simulink model "ConfiguredHevMmVirtualVehicle"  (R2025b)
settings: configuration reference "VehicleVariable" (kept outside this file)
StartFcn:
  | %tic
StopFcn:
  | %toc
model workspace (MAT data in the model file):
  ExtDrvCmdsSwitch : Simulink.Parameter (value not decoded)
  ExtDrvRefSwitch : Simulink.Parameter (value not decoded)
  ExtEnvSwitch : Simulink.Parameter (value not decoded)
  ExtGndSwitch : Simulink.Parameter (value not decoded)
symbols that are objects in the model workspace (value not decoded): ExtDrvCmdsSwitch, ExtDrvRefSwitch, ExtEnvSwitch, ExtGndSwitch
undefined symbols (not defined in the file or in its folder): AmbTemp, BaroPress, CurvGradRef, CurvRef, DCM, DriverAeroRes, DriverDrivelineRes, DriverInitialGear, DriverPreviewDist, DriverRollRes, DriverShiftTime, DriverTimeConst, DriverTractiveForce, EnvAbsPrs, EnvAirTemp, EnvGrvty, EnvNomFrictionScaling, EnvNominalGrade, EnvScnFrictionMap, EnvScnFrictionMapXBpts, EnvScnFrictionMapYBpts, EnvScnHeightMap, EnvScnHeightMapXBpts, EnvScnHeightMapYBpts, EnvWindVelX, EnvWindVelY, EnvWindVelZ, Gnd, Grade, HazzardCmd, HighBeamCmd, lambda_mux, LeftSignalCmd, LngRef, LowBeamCmd, LtrRef, PhiRef, PlntVehDstCGFrntAxl, PlntVehDstCGRearAxl, PlntVehInitLatPos, PlntVehInitLongPos, PlntVehInitPitchAng, PlntVehInitRollAng, PlntVehInitVertPos, PlntVehInitYawAng, PlntVehMass, PlntVehTrckWdth, PlntVehYawMomentInertia, PlntWhlLdRadiusFrnt, PlntWhlLdRadiusRear, RightSignalCmd, ScnCRRadius, Sim3dSensor, Wind, XRef, YRef, Z
libraries: simulink x28, autolibutils x8, autolibsharedcommon x7, vehdynlibscenariocommon x7, vehdynlibviscommon x4, vehdynlibdriver x2, sim3dgroundtruthsensorlib x2, sim3dlib x2, autolibshared x2, sim3dautolib x2, sl3dlib x1, sharedtransform x1
(part 4 of 6)

== system ConfiguredHevMmVirtualVehicle/Scenarios/Reference Generator/Constant Radius ==
  VehFdbk : Inport
  Bus Creator : BusCreator  Inputs=3
  Bus Selector : BusSelector  OutputSignals=Body.InertFrm.Geom.Disp.Z,Body.InertFrm.Geom.Disp.X,Body.InertFrm.Geom.Disp.Y,Body.InertFrm.Cg.Ang.psi
  Bus Selector1 : BusSelector  OutputSignals=XRef,YRef
  Constant Radius : vehdynlibscenariocommon/Constant Radius Signal Input  VariantControl=4  tStart=ScnStartTime  velRef=ScnLongVelRef  velRefUnit=mph  R=ScnCRRadius  X_o=PlntVehInitLongPos  Y_o=PlntVehInitLatPos  psi_o=PlntVehInitYawAng  radialConeDist=6  ayMax=ScnCRMaxLatAccel  steerDir=Right  ayStop=off  use3DCones=off  aMode=2
      settings: LibrarySourceBlock=vehdynlibscenario/Constant Radius
  Signal Copy : SignalConversion  OverrideOpt=off
  Signal Copy1 : SignalConversion  OverrideOpt=off
  Signal Copy2 : SignalConversion  OverrideOpt=off
  " Vis" : Outport
  DrvRef : Outport  Port=2  VectorParamsAs1DForOutWhenUnconnected=off
  DrvCmd : Outport  Port=3  VectorParamsAs1DForOutWhenUnconnected=off
  " Fdbk" : Outport  Port=4  VectorParamsAs1DForOutWhenUnconnected=off
  wires:
  VehFdbk/1 -> " Fdbk"/1, Bus Selector/1
  Bus Creator/1 -> " Vis"/1
  Constant Radius/2 -> DrvCmd/1
  Bus Selector/2 -> Constant Radius/1  "<X>"
  Bus Selector/3 -> Constant Radius/2  "<Y>"
  Bus Selector/4 -> Constant Radius/3  "<psi>"
  Constant Radius/1 -> Bus Selector1/1, DrvRef/1
  Bus Selector/1 -> Signal Copy/1  "<Z>"
  Signal Copy/1 -> Bus Creator/3  "ZRef"
  Signal Copy1/1 -> Bus Creator/2  "YRef"
  Signal Copy2/1 -> Bus Creator/1  "XRef"
  Bus Selector1/2 -> Signal Copy1/1  "<YRef>"
  Bus Selector1/1 -> Signal Copy2/1  "<XRef>"

== system ConfiguredHevMmVirtualVehicle/Scenarios/Reference Generator/Double Lane Change ==
  "VehFdbk " : Inport
  Bus Selector : BusSelector  OutputSignals=Body.BdyFrm.Cg.Vel.xdot,Body.InertFrm.Geom.Disp.X,Body.InertFrm.Geom.Disp.Y,Body.InertFrm.Cg.Ang.psi
  Double Lane Change : vehdynlibscenariocommon/Lane Change Signal Input  ssMode=Initialize from model  ssVar=dlcSS35mph  changeType=Obstacle avoidance (ISO 3888-2)  tStart=ScnStartTime  XGate=ScnDLCGateLongPos  velRef=ScnLongVelRef  velRefUnit=mph  xStart=ScnDLCLongRefStartPos  vehWidth=ScnDLCVehicleWidth  nomLatOffset=ScnDLCLatRefOffset  latRefbp=ScnDLCLongRefBpt  latRef=ScnDLCLatRef  centerSwitch=on  xSimStop=off  extInfo=on  use3DCones=off  ssDefault=on  X_o=0  Y_o=3.125  psi_o=0  ssTol=.1  ssMaxTime=30  ssWSName=dlcSS35mph  aMode=2
      settings: LibrarySourceBlock=vehdynlibscenario/Lane Change
  " Vis" : Outport  VectorParamsAs1DForOutWhenUnconnected=off
  DrvRef : Outport  Port=2  VectorParamsAs1DForOutWhenUnconnected=off
  DrvCmd : Outport  Port=3  VectorParamsAs1DForOutWhenUnconnected=off
  " Fdbk" : Outport  Port=4  VectorParamsAs1DForOutWhenUnconnected=off
  wires:
  "VehFdbk "/1 -> " Fdbk"/1, Bus Selector/1
  Double Lane Change/1 -> " Vis"/1
  Double Lane Change/2 -> DrvRef/1
  Bus Selector/1 -> Double Lane Change/1  "<xdot>"
  Double Lane Change/3 -> DrvCmd/1
  Bus Selector/2 -> Double Lane Change/2  "<X>"
  Bus Selector/3 -> Double Lane Change/3  "<Y>"
  Bus Selector/4 -> Double Lane Change/4  "<psi>"

== system ConfiguredHevMmVirtualVehicle/Scenarios/Reference Generator/Drive Cycle ==
  "VehFdbk " : Inport
  Bus Assignment : BusAssignment  AssignedSignals=LngRef,XRef
  Bus Creator : BusCreator  Inputs=3
  Bus Selector : BusSelector  OutputSignals=Body.InertFrm.Cg.Disp.X
  Constant13 : Constant  Value=0
  Constant14 : Constant  Value=0
  Constant15 : Constant  Value=0
  Drive Cycle Source : autolibshared/Drive Cycle Source  cycleVar=FTP75  fileVar=L:\Bauto\matlab\test\toolbox\shared\autoblks\scenario\adac.txt  tfinal="2474  seconds"  cycleRepeat=off  outAccPort=off  outGearPort=off  gearList=No gear data  t_wot1=t_start  xdot_woto=0  xdot_wot1=xdot_r  t_wot2=t_wot2  xdot_wot2=0  t_wotend=ScnSimTime  srcUnit=m/s  outUnit=mph  srcAccUnit=m/s/s  outAccUnit=m/s^2  dt=0  aMode=6  faultOption=off  velBnd=2  velBndUnit=mph  inUnit=m/s  timeBnd=1  failOption=off  stopSim=off  maxFaultCnt=10  maxFaultTime=2  maxTotFaultTime=15  traceOption=off  dtTrace=1  traceWindow=10  lastDCname=FTP75  lastOutUnit=mph  lastDT=0  lastTB=1  lastSB=2  forceCalcBound=off
  DrvCmdSrc : autolibsharedcommon/DrvCmd  SystemSampleTime=-1  VariantActivationTime=update diagram  EmptyChoice=off  PassThrough=off  PassThroughVariantControl=(default)  EmptyChoiceVariantControl=(default)  AllowFlexibleInterface=on  Latency=0  AutoFrameSizeCalculation=off
  DrvRefSrc : autolibsharedcommon/DrvRef  SystemSampleTime=-1  VariantActivationTime=update diagram  EmptyChoice=off  PassThrough=off  PassThroughVariantControl=(default)  EmptyChoiceVariantControl=(default)  AllowFlexibleInterface=on  Latency=0  AutoFrameSizeCalculation=off
  Unit Conversion : UnitConversion
  " Vis" : Outport  VectorParamsAs1DForOutWhenUnconnected=off
  DrvRef : Outport  Port=2  VectorParamsAs1DForOutWhenUnconnected=off
  DrvCmd : Outport  Port=3  VectorParamsAs1DForOutWhenUnconnected=off
  " Fdbk" : Outport  Port=4  VectorParamsAs1DForOutWhenUnconnected=off
  wires:
  Constant13/1 -> Bus Creator/1  "XRef"
  Constant14/1 -> Bus Creator/2  "YRef"
  Constant15/1 -> Bus Creator/3  "ZRef"
  Bus Creator/1 -> " Vis"/1
  Drive Cycle Source/1 -> Unit Conversion/1
  Bus Selector/1 -> Bus Assignment/3  "<X>"
  "VehFdbk "/1 -> Bus Selector/1, " Fdbk"/1
  DrvRefSrc/1 -> Bus Assignment/1
  Bus Assignment/1 -> DrvRef/1
  DrvCmdSrc/1 -> DrvCmd/1
  Unit Conversion/1 -> Bus Assignment/2

== system ConfiguredHevMmVirtualVehicle/Scenarios/Reference Generator/Fishhook ==
  "VehFdbk " : Inport
  Bus Creator : BusCreator  Inputs=3
  Bus Selector : BusSelector  OutputSignals=Body.BdyFrm.Cg.Vel.xdot
  Constant : Constant  Value=0
  Constant1 : Constant  Value=0
  Constant2 : Constant  Value=0
  Fishhook : vehdynlibscenariocommon/Fishhook Signal Input  ssMode=Initialize from model  ssVar=fh50mph  tStart=ScnStartTime  velRef=ScnLongVelRef  velRefUnit=mph  steerRate=ScnFHSteerSpeed  steerAmp=ScnFHSteerAmp  pFdbk=off  tDwellSteer=ScnFHInitialDwellTime  tDwellCntrSteer=ScnFHCounterDwellTime  tZero=ScnFHReturnTime  pZero=1.5  steerDir=Right  ssDefault=on  X_o=0  Y_o=0  psi_o=0  ssTol=.1  ssMaxTime=30  ssWSName=fh50mph  aMode=2
      settings: LibrarySourceBlock=vehdynlibscenario/Fishhook
  " Vis" : Outport  VectorParamsAs1DForOutWhenUnconnected=off
  DrvRef : Outport  Port=2  VectorParamsAs1DForOutWhenUnconnected=off
  DrvCmd : Outport  Port=3  VectorParamsAs1DForOutWhenUnconnected=off
  " Fdbk" : Outport  Port=4  VectorParamsAs1DForOutWhenUnconnected=off
  wires:
  Constant/1 -> Bus Creator/1  "XRef"
  Constant1/1 -> Bus Creator/2  "YRef"
  Constant2/1 -> Bus Creator/3  "ZRef"
  Bus Creator/1 -> " Vis"/1
  Fishhook/1 -> DrvRef/1
  Fishhook/2 -> DrvCmd/1
  "VehFdbk "/1 -> " Fdbk"/1, Bus Selector/1
  Bus Selector/1 -> Fishhook/1  "<xdot>"

== system ConfiguredHevMmVirtualVehicle/Scenarios/Reference Generator/Increasing Steer ==
  "VehFdbk " : Inport
  Bus Creator : BusCreator  Inputs=3
  Bus Selector : BusSelector  OutputSignals=Body.BdyFrm.Cg.Vel.xdot,Body.BdyFrm.Cg.Acc.ay
  Constant : Constant  Value=0
  Constant1 : Constant  Value=0
  Constant2 : Constant  Value=0
  Increasing Steer : vehdynlibscenariocommon/Increasing Steer Signal Input  ssMode=Initialize from model  ssVar=is50mph  tStart=ScnStartTime  velRef=ScnLongVelRef  velRefUnit=mph  steerRate=ScnISHandwheelRate  steerAmp=ScnISMaxHandwheelAng  tDwellSteer=ScnISSteerHoldTime  ayMax=ScnISMaxLatAccel  steerDir=Right  ayStop=on  ssDefault=on  X_o=0  Y_o=0  psi_o=0  ssTol=.1  ssMaxTime=30  ssWSName=is50mph  aMode=2
      settings: LibrarySourceBlock=vehdynlibscenario/Slowly Increasing Steer
  " Vis" : Outport  VectorParamsAs1DForOutWhenUnconnected=off
  DrvRef : Outport  Port=2  VectorParamsAs1DForOutWhenUnconnected=off
  DrvCmd : Outport  Port=3  VectorParamsAs1DForOutWhenUnconnected=off
  " Fdbk" : Outport  Port=4  VectorParamsAs1DForOutWhenUnconnected=off
  wires:
  "VehFdbk "/1 -> " Fdbk"/1, Bus Selector/1
  Bus Creator/1 -> " Vis"/1
  Constant2/1 -> Bus Creator/3  "ZRef"
  Constant1/1 -> Bus Creator/2  "YRef"
  Constant/1 -> Bus Creator/1  "XRef"
  Increasing Steer/1 -> DrvRef/1
  Increasing Steer/2 -> DrvCmd/1
  Bus Selector/1 -> Increasing Steer/1  "<xdot>"
  Bus Selector/2 -> Increasing Steer/2  "<ay>"

== system ConfiguredHevMmVirtualVehicle/Scenarios/Reference Generator/No Commands ==
  "VehFdbk " : Inport
  Bus Creator : BusCreator  Inputs=3
  Constant13 : Constant  Value=0
  Constant14 : Constant  Value=0
  Constant15 : Constant  Value=0
  DrvCmd1 : autolibsharedcommon/DrvCmd  SystemSampleTime=-1  VariantActivationTime=update diagram  EmptyChoice=off  PassThrough=off  PassThroughVariantControl=(default)  EmptyChoiceVariantControl=(default)  AllowFlexibleInterface=on  Latency=0  AutoFrameSizeCalculation=off
  DrvRef1 : autolibsharedcommon/DrvRef  SystemSampleTime=-1  VariantActivationTime=update diagram  EmptyChoice=off  PassThrough=off  PassThroughVariantControl=(default)  EmptyChoiceVariantControl=(default)  AllowFlexibleInterface=on  Latency=0  AutoFrameSizeCalculation=off
  Signal Specification4 : SignalSpecification  Unit=m
  Signal Specification5 : SignalSpecification  Unit=m
  Signal Specification6 : SignalSpecification  Unit=m
  " Vis" : Outport  VectorParamsAs1DForOutWhenUnconnected=off
  DrvRef : Outport  Port=2  VectorParamsAs1DForOutWhenUnconnected=off
  DrvCmd : Outport  Port=3  VectorParamsAs1DForOutWhenUnconnected=off
  " Fdbk" : Outport  Port=4  VectorParamsAs1DForOutWhenUnconnected=off
  wires:
  Signal Specification4/1 -> Bus Creator/1  "XRef"
  Signal Specification6/1 -> Bus Creator/3  "ZRef"
  Bus Creator/1 -> " Vis"/1
  "VehFdbk "/1 -> " Fdbk"/1
  Constant13/1 -> Signal Specification4/1
  Signal Specification5/1 -> Bus Creator/2  "YRef"
  Constant14/1 -> Signal Specification5/1
  Constant15/1 -> Signal Specification6/1
  DrvRef1/1 -> DrvRef/1
  DrvCmd1/1 -> DrvCmd/1

== system ConfiguredHevMmVirtualVehicle/Scenarios/Reference Generator/Sine with Dwell ==
  "VehFdbk " : Inport
  Bus Creator : BusCreator  Inputs=3
  Bus Selector : BusSelector  OutputSignals=Body.BdyFrm.Cg.Vel.xdot
  Constant : Constant  Value=0
  Constant1 : Constant  Value=0
  Constant2 : Constant  Value=0
  Sine with Dwell : vehdynlibscenariocommon/Sine With Dwell Signal Input  ssMode=Initialize from model  ssVar=swd50mph  tStart=ScnStartTime  velRef=ScnLongVelRef  velRefUnit=mph  steerFreq=ScnSDSteerFreq  steerAmp=ScnSDSteerAmp  tDwellCntrSteer=ScnSDDwellTime  steerDir=Right  ssDefault=on  X_o=0  Y_o=0  psi_o=0  ssTol=.1  ssMaxTime=30  ssWSName=swd50mph  aMode=2
      settings: LibrarySourceBlock=vehdynlibscenario/Sine With Dwell
  " Vis" : Outport  VectorParamsAs1DForOutWhenUnconnected=off
  DrvRef : Outport  Port=2  VectorParamsAs1DForOutWhenUnconnected=off
  DrvCmd : Outport  Port=3  VectorParamsAs1DForOutWhenUnconnected=off
  " Fdbk" : Outport  Port=4  VectorParamsAs1DForOutWhenUnconnected=off
  wires:
  "VehFdbk "/1 -> " Fdbk"/1, Bus Selector/1
  Bus Creator/1 -> " Vis"/1
  Constant2/1 -> Bus Creator/3  "ZRef"
  Constant1/1 -> Bus Creator/2  "YRef"
  Constant/1 -> Bus Creator/1  "XRef"
  Sine with Dwell/1 -> DrvRef/1
  Sine with Dwell/2 -> DrvCmd/1
  Bus Selector/1 -> Sine with Dwell/1  "<xdot>"

== system ConfiguredHevMmVirtualVehicle/Scenarios/Reference Generator/Swept Sine ==
  "VehFdbk " : Inport
  Bus Creator : BusCreator  Inputs=3
  Bus Selector : BusSelector  OutputSignals=Body.BdyFrm.Cg.Vel.xdot
  Constant : Constant  Value=0
  Constant1 : Constant  Value=0
  Constant2 : Constant  Value=0
  Swept Sine : vehdynlibscenariocommon/Swept Sine Signal Input  ssMode=Initialize from model  ssVar=ss30mph  tStart=ScnStartTime  velRef=ScnLongVelRef  velRefUnit=mph  steerAmp=ScnSSSteerAmp  steerFinalFreq=ScnSSFinalFreq  tSweep=ScnSSSweepTime  ssDefault=on  steerDir=Right  X_o=0  Y_o=0  psi_o=0  ssTol=.1  ssMaxTime=30  ssWSName=ss30mph  aMode=2
      settings: LibrarySourceBlock=vehdynlibscenario/Swept Sine
  " Vis" : Outport  VectorParamsAs1DForOutWhenUnconnected=off
  DrvRef : Outport  Port=2  VectorParamsAs1DForOutWhenUnconnected=off
  DrvCmd : Outport  Port=3  VectorParamsAs1DForOutWhenUnconnected=off
  " Fdbk" : Outport  Port=4  VectorParamsAs1DForOutWhenUnconnected=off
  wires:
  "VehFdbk "/1 -> " Fdbk"/1, Bus Selector/1
  Bus Creator/1 -> " Vis"/1
  Constant2/1 -> Bus Creator/3  "ZRef"
  Constant1/1 -> Bus Creator/2  "YRef"
  Constant/1 -> Bus Creator/1  "XRef"
  Bus Selector/1 -> Swept Sine/1  "<xdot>"
  Swept Sine/1 -> DrvRef/1
  Swept Sine/2 -> DrvCmd/1

== system ConfiguredHevMmVirtualVehicle/Scenarios/Reference Generator/WOT ==
  "VehFdbk " : Inport
  Bus Assignment : BusAssignment  AssignedSignals=LngRef,XRef,YRef,PhiRef
  Bus Creator : BusCreator  Inputs=3
  Bus Selector : BusSelector  OutputSignals=Body.InertFrm.Cg.Disp.X,Body.InertFrm.Cg.Disp.Y,Body.InertFrm.Cg.Ang.psi
  Constant13 : Constant  Value=0
  Constant14 : Constant  Value=0
  Constant15 : Constant  Value=0
  Drive Cycle Source : autolibshared/Drive Cycle Source  cycleVar=Wide Open Throttle (WOT)  fileVar=L:\Bauto\matlab\test\toolbox\shared\autoblks\scenario\adac.txt  tfinal="40  seconds"  cycleRepeat=off  outAccPort=off  outGearPort=off  gearList=No gear data  t_wot1=ScnStartTime  xdot_woto=0  xdot_wot1=ScnLongVelRef  t_wot2=ScnTimeToStrtDecel  xdot_wot2=0  t_wotend=40  srcUnit=mph  outUnit=mph  srcAccUnit=m/s/s  outAccUnit=m/s^2  dt=0  aMode=6  faultOption=off  velBnd=2  velBndUnit=mph  inUnit=m/s  timeBnd=1  failOption=off  stopSim=off  maxFaultCnt=10  maxFaultTime=2  maxTotFaultTime=15  traceOption=off  dtTrace=1  traceWindow=10  lastDCname=Custom Data Set  lastOutUnit=mph  lastDT=0  lastTB=1  lastSB=2  forceCalcBound=off
  DrvCmdSrc : autolibsharedcommon/DrvCmd  SystemSampleTime=-1  VariantActivationTime=update diagram  EmptyChoice=off  PassThrough=off  PassThroughVariantControl=(default)  EmptyChoiceVariantControl=(default)  AllowFlexibleInterface=on  Latency=0  AutoFrameSizeCalculation=off
  DrvRefSrc : autolibsharedcommon/DrvRef  SystemSampleTime=-1  VariantActivationTime=update diagram  EmptyChoice=off  PassThrough=off  PassThroughVariantControl=(default)  EmptyChoiceVariantControl=(default)  AllowFlexibleInterface=on  Latency=0  AutoFrameSizeCalculation=off
  Unit Conversion : UnitConversion
  " Vis" : Outport  VectorParamsAs1DForOutWhenUnconnected=off
  " Fdbk" : Outport  Port=2  VectorParamsAs1DForOutWhenUnconnected=off
  DrvRef : Outport  Port=3  VectorParamsAs1DForOutWhenUnconnected=off
  DrvCmd : Outport  Port=4  VectorParamsAs1DForOutWhenUnconnected=off
  wires:
  Drive Cycle Source/1 -> Unit Conversion/1
  Bus Creator/1 -> " Vis"/1
  Constant15/1 -> Bus Creator/3  "ZRef"
  Constant14/1 -> Bus Creator/2  "YRef"
  Constant13/1 -> Bus Creator/1  "XRef"
  Bus Selector/2 -> Bus Assignment/4  "<Y>"
  DrvRefSrc/1 -> Bus Assignment/1
  DrvCmdSrc/1 -> DrvCmd/1
  Bus Selector/1 -> Bus Assignment/3  "<X>"
  Bus Assignment/1 -> DrvRef/1
  Bus Selector/3 -> Bus Assignment/5  "<psi>"
  "VehFdbk "/1 -> Bus Selector/1, " Fdbk"/1
  Unit Conversion/1 -> Bus Assignment/2

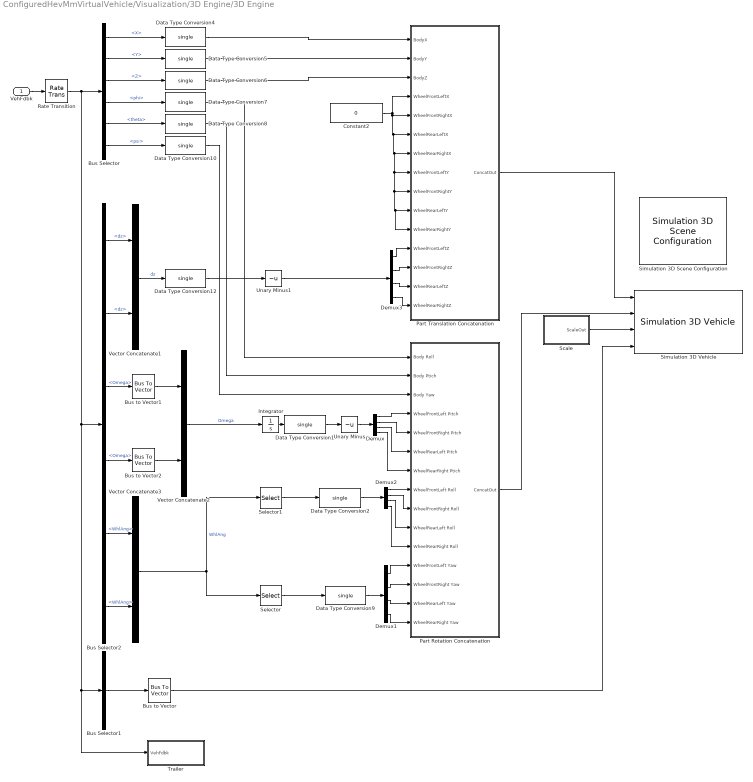
== system ConfiguredHevMmVirtualVehicle/Visualization/3D Engine/3D Engine ==
  VehFdbk : Inport
  Bus Selector : BusSelector  OutputSignals=Body.InertFrm.Geom.Disp.X,Body.InertFrm.Geom.Disp.Y,Body.InertFrm.Geom.Disp.Z,Body.InertFrm.Cg.Ang.phi,Body.InertFrm.Cg.Ang.theta,Body.InertFrm.Cg.Ang.psi
  Bus Selector1 : BusSelector  OutputSignals=Driver.LightsFdbk.HighBeamFdbk,Driver.LightsFdbk.LowBeamFdbk,Driver.LightsFdbk.BrakeLightFdbk,Driver.LightsFdbk.ReverseLightFdbk,Driver.LightsFdbk.LeftSignalFdbk,Driver.LightsFdbk.RightSignalFdbk  OutputAsBus=on
  Bus Selector2 : BusSelector  OutputSignals=FrntSuspension.FrntSuspWheel.dz,RearSuspension.RearSuspWheel.dz,FrntWheels.Wheels.Omega,RearWheels.Wheels.Omega,FrntSuspension.FrntSuspWheel.WhlAng,RearSuspension.RearSuspWheel.WhlAng
  Bus to Vector : BusToVector
  Bus to Vector1 : BusToVector
  Bus to Vector2 : BusToVector
  Constant2 : Constant  Value=0  OutDataTypeStr=single
  Data Type Conversion{1..2,4..10,12} (10 alike) : DataTypeConversion  OutDataTypeStr=single  SaturateOnIntegerOverflow=off  RndMeth=Floor
  Demux{,1..3} (4 alike) : Demux
  Integrator : Integrator  WrapState=on  WrappedStateUpperValue=2*pi  WrappedStateLowerValue=0  ZeroCross=off
  Part Rotation Concatenation : Subsystem
  Part Translation Concatenation : Subsystem
  Rate Transition : RateTransition  OutPortSampleTime=0.03
  Scale : Subsystem
  Selector : Selector  NumberOfDimensions=2  InputPortWidth=3  IndexOptions=Index vector (dialog),Select all  Indices=[3],1  OutputSizes=1,1
  Selector1 : Selector  NumberOfDimensions=2  InputPortWidth=3  IndexOptions=Index vector (dialog),Select all  Indices=[1],1  OutputSizes=1,1
  Simulation 3D Scene Configuration : sim3dlib/Simulation 3D Scene Configuration  Priority=0  ProjectFormat=Default Scenes  SceneDesc=Open surface  ProjectName=/mathworks/devel/bat/filer/batfs2552-0/BR2025bd.2978516/build/matlab/toolbox/shared/sim3d_projects/automotive_project_linux/UE/LinuxNoEditor/VehicleSimulation.sh  ScenePath=/Game/Maps/HwStrght  EnableOpenDRIVE=off  vehTagList={'Custom';'Scene Origin';'SimulinkVehicle1'}  vehTag=SimulinkVehicle1  AttachedCameraRelativeTranslation=[0 0 0]  FreeCameraDefaultInitialTranslation=[-6, 0, 2]  AttachedCameraRelativeRotation=[0 0 0]  FreeCameraDefaultInitialRotation=[0, -15, 0]  ViewpointName=Custom  FreeCameraInitialTranslation=[0 0 0]  ViewpointTranslation=[0 0 0]  FreeCameraInitialRotation=[0 0 0]  ViewpointRotation=[0 0 0]  OpVisEn=off  Ts=0.03  EnableWindow=on  EnableRemoteAccess=off  EnableWeather=off  SunAzimuth=90  SunAltitude=40.0  EnableGeospatialSun=off  Latitude=0  Longitude=0  Date=2023-01-01  Time=10:30:00  GeoTimeZone=-5.0  SunDaylightSaving=off  wind=1  clouds=10  EnableVolumetricClouds=off  CloudCoverage=0  CloudAltitude=6  fog=0  rain=0  RaindropsEffect=off  SnowDensity=0  EnableGeospatial=off  TilesetSource=Earth terrain  UseTrueOrigin=off  OriginHeight=200  OriginLatitude=40.744652  OriginLongitude=-73.988864  MapStyle=Aerial  AdditionalAssetIDs=[]  UseAdvancedSunSky=off  SolarTime=11  TimeZone=-5  Day=21  Month=9  Year=2022  UseDaylightSavingTime=on  DSTStartDay=10  DSTStartMonth=3  DSTEndDay=3  DSTEndMonth=11  DSTSwitchHour=2  sensorTag=MainCamera4  sensorId=4  sensorName=MainCamera4  mountLoc=Origin  offsetFlag=off  tmountOffset=[0, 0, 0]  rmountOffset=[0, 0, 0]  HorizontalResolution=1280  VerticalResolution=720  HorizontalFOV=60  mountPoint=[0 0 0]  mountOrientation=[0 0 0]  aMode=2  ID=4  GeoTrigger=Inactive  ViewNameList={'Custom'}  ViewTranslationList={'[0 0 0]'}  ViewRotationList={'[0 0 0]'}
      settings: LibrarySourceBlock=vdynlib/Vehicle Scenarios/Sim3D/Sim3D Core/Simulation 3D Scene Configuration
  Simulation 3D Vehicle : sim3dautolib/Simulation 3D Vehicle  Priority=-1  PassVehMesh=Muscle car  MeshPath=/MathWorksSimulation/Vehicles/Muscle/Meshes/SK_MuscleCar.SK_MuscleCar  VehColor=Red  ActorName=SimulinkVehicle1  VehLightsControl=on  HeadlightColor=[ 1, 1, 1 ]  HighBeamIntensity=100000  LowBeamIntensity=60000  HighBeamConeAngle=1.22  LowBeamConeAngle=1.22  LeftHeadlightOrientation=[ 0, 0 ]  RightHeadlightOrientation=[ 0, 0 ]  BrakelightIntensity=500  ReverselightIntensity=500  SignallightIntensity=500  SignallightPeriod=1  SignalPulseWidth=50  Translation=[PlntVehInitLongPos PlntVehInitLatPos -PlntVehInitVertPos; 0 0 0; 0 0 0; 0 0 0; 0 0 0]  Rotation=[PlntVehInitRollAng PlntVehInitPitchAng PlntVehInitYawAng; 0 0 0; 0 0 0; 0 0 0; 0 0 0]  Scale=ones( 5, 3 )  SampleTime=0.03  ActorType=SimulinkVehicle  ID=1  aMode=2  ActorTag=SimulinkVehicle1
  Trailer : Subsystem  Variant=on  VariantControlMode=label  LabelModeActiveChoice=No Trailer
  Unary Minus : UnaryMinus
  Unary Minus1 : UnaryMinus
  Vector Concatenate1 : Concatenate
  Vector Concatenate2 : Concatenate
  Vector Concatenate3 : Concatenate  Mode=Multidimensional array  ConcatenateDimension=2
  wires:
  Data Type Conversion7/1 -> Part Rotation Concatenation/1(Body Roll)
  Constant2/1 -> Part Translation Concatenation/4(WheelFrontLeftX), Part Translation Concatenation/11(WheelRearRightY), Part Translation Concatenation/10(WheelRearLeftY), Part Translation Concatenation/9(WheelFrontRightY), Part Translation Concatenation/8(WheelFrontLeftY), Part Translation Concatenation/7(WheelRearRightX), Part Translation Concatenation/6(WheelRearLeftX), Part Translation Concatenation/5(WheelFrontRightX)
  Data Type Conversion8/1 -> Part Rotation Concatenation/2(Body Ptich)
  Bus Selector2/4 -> Bus to Vector2/1  "<Omega>"
  Bus Selector2/5 -> Vector Concatenate3/1  "<WhlAng>"
  Data Type Conversion10/1 -> Part Rotation Concatenation/3(Body Yaw)
  Demux1/4 -> Part Rotation Concatenation/15(WheelRearRight Yaw)
  VehFdbk/1 -> Rate Transition/1
  Vector Concatenate3/1 -> Selector1/1, Selector/1  "WhlAng"
  Vector Concatenate2/1 -> Integrator/1  "Omega"
  Demux2/1 -> Part Rotation Concatenation/8(WheelFrontLeft Roll)
  Demux/1 -> Part Rotation Concatenation/4(WheelFrontLeft Pitch)
  Demux/2 -> Part Rotation Concatenation/5(WheelFrontRight Pitch)
  Demux3/2 -> Part Translation Concatenation/13(WheelFrontRightZ)
  Demux/3 -> Part Rotation Concatenation/6(WheelRearLeft Pitch)
  Part Rotation Concatenation/1(ConcatOut) -> Simulation 3D Vehicle/2
  Demux2/3 -> Part Rotation Concatenation/10(WheelRearLeft Roll)
  Demux1/1 -> Part Rotation Concatenation/12(WheelFrontLeft Yaw)
  Demux/4 -> Part Rotation Concatenation/7(WheelRearRight Ptich)
  Bus Selector2/2 -> Vector Concatenate1/2  "<dz>"
  Data Type Conversion6/1 -> Part Translation Concatenation/3(BodyZ)
  Bus Selector/6 -> Data Type Conversion10/1  "<psi>"
  Bus Selector/5 -> Data Type Conversion8/1  "<theta>"
  Bus to Vector1/1 -> Vector Concatenate2/1
  Demux3/4 -> Part Translation Concatenation/15(WheelRearRightZ)
  Bus Selector/2 -> Data Type Conversion5/1  "<Y>"
  Demux1/2 -> Part Rotation Concatenation/13(WheelFrontRight Yaw)
  Data Type Conversion5/1 -> Part Translation Concatenation/2(BodyY)
  Data Type Conversion12/1 -> Unary Minus1/1
  Bus Selector/4 -> Data Type Conversion7/1  "<phi>"
  Selector/1 -> Data Type Conversion9/1
  Bus Selector2/1 -> Vector Concatenate1/1  "<dz>"
  Bus to Vector2/1 -> Vector Concatenate2/2
  Data Type Conversion1/1 -> Unary Minus/1
  Data Type Conversion4/1 -> Part Translation Concatenation/1(BodyX)
  Data Type Conversion2/1 -> Demux2/1
  Selector1/1 -> Data Type Conversion2/1
  Bus Selector/3 -> Data Type Conversion6/1  "<Z>"
  Part Translation Concatenation/1(ConcatOut) -> Simulation 3D Vehicle/1
  Bus Selector2/3 -> Bus to Vector1/1  "<Omega>"
  Demux3/3 -> Part Translation Concatenation/14(WheelRearLeftZ)
  Unary Minus/1 -> Demux/1
  Rate Transition/1 -> Trailer/1(VehFdbk), Bus Selector1/1, Bus Selector2/1, Bus Selector/1
  Bus to Vector/1 -> Simulation 3D Vehicle/4
  Demux2/4 -> Part Rotation Concatenation/11(WheelRearRight Roll)
  Integrator/1 -> Data Type Conversion1/1
  Data Type Conversion9/1 -> Demux1/1
  Bus Selector1/1 -> Bus to Vector/1
  Demux2/2 -> Part Rotation Concatenation/9(WheelFrontRight Roll)
  Unary Minus1/1 -> Demux3/1
  Vector Concatenate1/1 -> Data Type Conversion12/1  "dz"
  Bus Selector/1 -> Data Type Conversion4/1  "<X>"
  Demux3/1 -> Part Translation Concatenation/12(WheelFrontLeftZ)
  Demux1/3 -> Part Rotation Concatenation/14(WheelRearLeft Yaw)
  Scale/1(ScaleOut) -> Simulation 3D Vehicle/3
  Bus Selector2/6 -> Vector Concatenate3/2  "<WhlAng>"

== system ConfiguredHevMmVirtualVehicle/Visualization/3D Engine/3D Engine Disabled ==
  VehFdbk : Inport
  Terminator : Terminator
  wires:
  VehFdbk/1 -> Terminator/1

== system ConfiguredHevMmVirtualVehicle/Visualization/Coordinate Systems/ISO 8855 (Z-up) ==
  VehFdbkIn : Inport
  Bus Assignment : BusAssignment  AssignedSignals=Body.InertFrm.Cg.Disp.Y,Body.InertFrm.Cg.Disp.Z,Body.InertFrm.Cg.Vel.Ydot,Body.InertFrm.Cg.Vel.Zdot,Body.InertFrm.Geom.Disp.Y,Body.InertFrm.Geom.Disp.Z,Body.InertFrm.Cg.Ang.theta,Body.InertFrm.Cg.Ang.psi,Body.BdyFrm.Cg.Vel.ydot,Body.BdyFrm.Cg.Vel.zdot,Body.BdyFrm.Cg.AngVel.q,Body.BdyFrm.Cg.AngVel.r,Body.BdyFrm.Cg.Acc.ay,Body.BdyFrm.Cg.Acc.az,Body.BdyFrm.Cg.Acc.yddot,Body.BdyFrm.Cg.Acc.zddot
  Bus Selector : BusSelector  OutputSignals=Body.InertFrm.Cg.Disp.Y,Body.InertFrm.Cg.Disp.Z,Body.InertFrm.Cg.Vel.Ydot,Body.InertFrm.Cg.Vel.Zdot,Body.InertFrm.Geom.Disp.Y,Body.InertFrm.Geom.Disp.Z,Body.InertFrm.Cg.Ang.theta,Body.InertFrm.Cg.Ang.psi,Body.BdyFrm.Cg.Vel.ydot,Body.BdyFrm.Cg.Vel.zdot,Body.BdyFrm.Cg.AngVel.q,Body.BdyFrm.Cg.AngVel.r,Body.BdyFrm.Cg.Acc.ay,Body.BdyFrm.Cg.Acc.az,Body.BdyFrm.Cg.Acc.yddot,Body.BdyFrm.Cg.Acc.zddot
  Unary Minus{,1..15} (16 alike) : UnaryMinus
  VehFdbk : Outport
  wires:
  VehFdbkIn/1 -> Bus Assignment/1, Bus Selector/1
  Bus Assignment/1 -> VehFdbk/1
  Bus Selector/1 -> Unary Minus/1  "<Y>"
  Bus Selector/2 -> Unary Minus2/1  "<Z>"
  Bus Selector/11 -> Unary Minus10/1  "<q>"
  Bus Selector/12 -> Unary Minus11/1  "<r>"
  Bus Selector/13 -> Unary Minus12/1  "<ay>"
  Bus Selector/14 -> Unary Minus13/1  "<az>"
  Bus Selector/15 -> Unary Minus14/1  "<yddot>"
  Bus Selector/16 -> Unary Minus15/1  "<zddot>"
  Bus Selector/3 -> Unary Minus3/1  "<Ydot>"
  Bus Selector/4 -> Unary Minus4/1  "<Zdot>"
  Bus Selector/5 -> Unary Minus5/1  "<Y>"
  Bus Selector/6 -> Unary Minus1/1  "<Z>"
  Bus Selector/7 -> Unary Minus6/1  "<theta>"
  Bus Selector/8 -> Unary Minus7/1  "<psi>"
  Bus Selector/9 -> Unary Minus8/1  "<ydot>"
  Bus Selector/10 -> Unary Minus9/1  "<zdot>"
  Unary Minus/1 -> Bus Assignment/2
  Unary Minus2/1 -> Bus Assignment/3
  Unary Minus3/1 -> Bus Assignment/4
  Unary Minus4/1 -> Bus Assignment/5
  Unary Minus8/1 -> Bus Assignment/10
  Unary Minus9/1 -> Bus Assignment/11
  Unary Minus10/1 -> Bus Assignment/12
  Unary Minus11/1 -> Bus Assignment/13
  Unary Minus12/1 -> Bus Assignment/14
  Unary Minus13/1 -> Bus Assignment/15
  Unary Minus14/1 -> Bus Assignment/16
  Unary Minus15/1 -> Bus Assignment/17
  Unary Minus5/1 -> Bus Assignment/6
  Unary Minus1/1 -> Bus Assignment/7
  Unary Minus6/1 -> Bus Assignment/8
  Unary Minus7/1 -> Bus Assignment/9

== system ConfiguredHevMmVirtualVehicle/Visualization/Coordinate Systems/SAE J670 (Z-down) ==
  VehFdbkIn : Inport
  VehFdbk : Outport
  wires:
  VehFdbkIn/1 -> VehFdbk/1

== system ConfiguredHevMmVirtualVehicle/Visualization/ISO 15037-1:2006/Disabled ==
  VehFdbk : Inport
  Terminator1 : Terminator
  wires:
  VehFdbk/1 -> Terminator1/1

== system ConfiguredHevMmVirtualVehicle/Visualization/ISO 15037-1:2006/Enabled ==
  VehFdbk : Inport
  Bus Selector : BusSelector  OutputSignals=Driver.SteerFdbk,Body.BdyFrm.Cg.Vel.xdot,Body.BdyFrm.Cg.Vel.ydot,Body.BdyFrm.Cg.Acc.ax,Body.BdyFrm.Cg.Acc.ay,Body.BdyFrm.Cg.AngVel.r,Body.BdyFrm.Cg.AngVel.q,Body.BdyFrm.Cg.AngVel.p,Body.InertFrm.Cg.Ang.phi,Body.InertFrm.Cg.Ang.theta
  Signal Specification : SignalSpecification  Unit=deg
  Signal Specification10 : SignalSpecification  Unit=deg
  Signal Specification11 : SignalSpecification  Unit=deg
  Signal Specification2 : SignalSpecification  Unit=km/h
  Signal Specification3 : SignalSpecification  Unit=m/s
  Signal Specification5 : SignalSpecification  Unit=m/s^2
  Signal Specification6 : SignalSpecification  Unit=m/s^2
  Signal Specification7 : SignalSpecification  Unit=deg/s
  Signal Specification8 : SignalSpecification  Unit=deg/s
  Signal Specification9 : SignalSpecification  Unit=deg/s
  Terminator{,2..3,5..11} (10 alike) : Terminator
  Unit Conversion{2..4,6..12} (10 alike) : UnitConversion
  wires:
  Bus Selector/10 -> Unit Conversion12/1  "<theta>"
  Signal Specification11/1 -> Terminator11/1  "Pitch angle"
  Unit Conversion12/1 -> Signal Specification11/1
  Bus Selector/9 -> Unit Conversion11/1  "<phi>"
  Unit Conversion11/1 -> Signal Specification10/1
  Signal Specification10/1 -> Terminator10/1  "Roll angle"
  Bus Selector/8 -> Unit Conversion10/1  "<p>"
  Signal Specification9/1 -> Terminator9/1  "Roll velocity"
  Unit Conversion10/1 -> Signal Specification9/1
  Bus Selector/7 -> Unit Conversion9/1  "<q>"
  Unit Conversion9/1 -> Signal Specification8/1
  Signal Specification8/1 -> Terminator8/1  "Pitch velocity"
  Bus Selector/6 -> Unit Conversion8/1  "<r>"
  Signal Specification7/1 -> Terminator7/1  "Yaw velocity"
  Unit Conversion8/1 -> Signal Specification7/1
  Bus Selector/5 -> Unit Conversion7/1  "<ay>"
  Unit Conversion7/1 -> Signal Specification6/1
  Signal Specification6/1 -> Terminator6/1  "Lateral acceleration"
  Bus Selector/4 -> Unit Conversion6/1  "<ax>"
  Signal Specification5/1 -> Terminator5/1  "Longitudinal acceleration"
  Unit Conversion6/1 -> Signal Specification5/1
  Bus Selector/3 -> Unit Conversion4/1  "<ydot>"
  Signal Specification3/1 -> Terminator3/1  "Lateral velocity"
  Unit Conversion4/1 -> Signal Specification3/1
  Bus Selector/2 -> Unit Conversion3/1  "<xdot>"
  Unit Conversion3/1 -> Signal Specification2/1
  Signal Specification2/1 -> Terminator2/1  "Longitudinal velocity"
  Signal Specification/1 -> Terminator/1  "Steering-wheel angle"
  Unit Conversion2/1 -> Signal Specification/1
  VehFdbk/1 -> Bus Selector/1
  Bus Selector/1 -> Unit Conversion2/1  "<SteerFdbk>"

== system ConfiguredHevMmVirtualVehicle/Visualization/Scope Type/DLC ==
  VehFdbk : Inport
  Vis : Inport  Port=2
  Bus Creator : BusCreator  Inputs=3
  Bus Selector3 : BusSelector  OutputSignals=Body.InertFrm.Cg.Disp.X,Body.InertFrm.Cg.Disp.Z
  Bus Selector4 : BusSelector  OutputSignals=LeftBnd,RightBnd,LtrlRef
  Lane Change : Scope
      settings: Title=Double Lane Change: Lateral Displacement  ActiveDisplayYMinimum=-3.28469  ActiveDisplayYMaximum=6.06905  YLabel=Lateral Displacement [m] (positive = right direction)  DataLoggingSaveFormat=Array
  Mux1 : Mux  Inputs=3
  Rate Transition : RateTransition  OutPortSampleTime=.1
  Rate Transition1 : RateTransition  OutPortSampleTime=.1
  Rate Transition3 : RateTransition  OutPortSampleTime=.1
  Signal Copy : SignalConversion  OverrideOpt=off
  Signal Copy1 : SignalConversion  OverrideOpt=off
  Signal Copy2 : SignalConversion  OverrideOpt=off
  Ref : Outport  VectorParamsAs1DForOutWhenUnconnected=off
  wires:
  VehFdbk/1 -> Bus Selector3/1
  Vis/1 -> Bus Selector4/1
  Bus Creator/1 -> Ref/1
  Bus Selector3/2 -> Signal Copy2/1  "<Z>"
  Signal Copy/1 -> Bus Creator/2  "YRef"
  Signal Copy1/1 -> Bus Creator/1  "XRef"
  Signal Copy2/1 -> Bus Creator/3  "ZRef"
  Rate Transition3/1 -> Mux1/2  "Right Boundary"
  Bus Selector4/3 -> Signal Copy/1, Rate Transition1/1  "<LtrlRef>"
  Mux1/1 -> Lane Change/1
  Bus Selector4/1 -> Rate Transition/1  "<LeftBnd>"
  Rate Transition/1 -> Mux1/1  "Left Boundary"
  Bus Selector4/2 -> Rate Transition3/1  "<RightBnd>"
  Bus Selector3/1 -> Signal Copy1/1  "<X>"
  Rate Transition1/1 -> Mux1/3  "Reference"

== system ConfiguredHevMmVirtualVehicle/Visualization/Scope Type/None ==
  VehFdbk : Inport
  Vis : Inport  Port=2
  Bus Selector2 : BusSelector  OutputSignals=Driver.SteerFdbk
  Bus Selector9 : BusSelector  OutputSignals=Body.BdyFrm.Cg.AngVel.r
  Signal Specification1 : SignalSpecification  Unit=rad/s
  Signal Specification3 : SignalSpecification  Unit=deg/s
  Unit Conversion4 : UnitConversion
  Yaw Rate and Steer : Scope  NumInputPorts=2
      settings: ActiveDisplayYMinimum=-112.49987  ActiveDisplayYMaximum=112.49996
  Ref : Outport  VectorParamsAs1DForOutWhenUnconnected=off
  wires:
  Bus Selector9/1 -> Signal Specification1/1  "<r>"
  Signal Specification3/1 -> Yaw Rate and Steer/1
  Unit Conversion4/1 -> Signal Specification3/1
  VehFdbk/1 -> Bus Selector2/1, Bus Selector9/1  "VehFdbk"
  Bus Selector2/1 -> Yaw Rate and Steer/2  "<SteerFdbk>"
  Vis/1 -> Ref/1
  Signal Specification1/1 -> Unit Conversion4/1

== system ConfiguredHevMmVirtualVehicle/Visualization/Scope Type/XYZ ==
  VehFdbk : Inport
  Vis : Inport  Port=2
  Terminator : Terminator
  Ref : Outport  VectorParamsAs1DForOutWhenUnconnected=off
  wires:
  Vis/1 -> Ref/1
  VehFdbk/1 -> Terminator/1

== system ConfiguredHevMmVirtualVehicle/Visualization/Vehicle XY Plotter/Disabled ==

== system ConfiguredHevMmVirtualVehicle/Visualization/Vehicle XY Plotter/XY View ==
  Bus Element In2 : Inport  PortName=VehFdbk
  Bus Selector1 : BusSelector  OutputSignals=Body.InertFrm.Cg.Ang.phi,Body.InertFrm.Cg.Ang.theta,Body.InertFrm.Cg.Ang.psi  OutputAsBus=on
  Bus Selector10 : BusSelector  OutputSignals=FrntWheels.Wheels.Fx,RearWheels.Wheels.Fx,FrntWheels.Wheels.Fy,RearWheels.Wheels.Fy
  Bus Selector5 : BusSelector  OutputSignals=Steering.Front.WhlAng.FL,Steering.Front.WhlAng.FR,Steering.Rear.WhlAng.RL,Steering.Rear.WhlAng.RR  OutputAsBus=on
  Bus Selector6 : BusSelector  OutputSignals=Body.InertFrm.Geom.Disp.X,Body.InertFrm.Geom.Disp.Y,Body.InertFrm.Geom.Disp.Z  OutputAsBus=on
  Bus Selector7 : BusSelector  OutputSignals=Body.InertFrm.Geom.Vel.Xdot,Body.InertFrm.Geom.Vel.Ydot,Body.InertFrm.Geom.Vel.Zdot  OutputAsBus=on
  Bus Selector9 : BusSelector  OutputSignals=Trans.Info.Eng.EngSpd,EM.EMSpd,Trans.Info.Trans.TransGear
  Bus to Vector{,1..2,4..6} (6 alike) : BusToVector
  Driveline Speed : Subsystem
  Vector Concatenate : Concatenate
  Vector Concatenate1 : Concatenate
  Vector Concatenate2 : Concatenate
  Vehicle XY Plotter : vehdynlibviscommon/Vehicle XY Plot Configuration  extRef=off  extStats=on  extTireF=on  a=PlntVehDstCGFrntAxl  b=PlntVehDstCGRearAxl  w=PlntVehTrckWdth(1)  figBorder=10  bufferSize=1024  velNorm=5  tireFNorm=1000  pltDT=.1
  wires:
  Bus Selector7/1 -> Bus to Vector1/1
  Bus Selector5/1 -> Bus to Vector4/1
  Bus to Vector1/1 -> Vehicle XY Plotter/3
  Bus Selector1/1 -> Bus to Vector2/1
  Vector Concatenate2/1 -> Vehicle XY Plotter/5
  Bus to Vector/1 -> Vehicle XY Plotter/1
  Bus Selector6/1 -> Bus to Vector/1
  Bus to Vector2/1 -> Vehicle XY Plotter/2
  Bus Element In2/1 -> Bus Selector5/1, Bus Selector10/1, Bus Selector9/1, Bus Selector7/1, Bus Selector1/1, Bus Selector6/1  "VehFdbk"
  Bus to Vector4/1 -> Vehicle XY Plotter/4
  Bus Selector10/2 -> Bus to Vector6/1  "<Fx>"
  Vector Concatenate1/1 -> Vehicle XY Plotter/7
  Vector Concatenate/1 -> Vehicle XY Plotter/6
  Bus Selector10/1 -> Bus to Vector5/1  "<Fx>"
  Bus Selector10/3 -> Vector Concatenate1/1  "<Fy>"
  Bus Selector10/4 -> Vector Concatenate1/2  "<Fy>"
  Bus to Vector5/1 -> Vector Concatenate/1
  Bus to Vector6/1 -> Vector Concatenate/2
  Bus Selector9/3 -> Vector Concatenate2/2  "<TransGear>"
  Bus Selector9/2 -> Driveline Speed/2(<EMSpd>)  "<EMSpd>"
  Driveline Speed/1(MaxSpd) -> Vector Concatenate2/1
  Bus Selector9/1 -> Driveline Speed/1(<EngSpd>)  "<EngSpd>"

== system ConfiguredHevMmVirtualVehicle/Visualization/Vehicle XY Plotter/XY View Ref ==
  Bus Element In2 : Inport  PortName=VehFdbk
  Bus Element In1 : Inport  Port=2  PortName=Ref  Element=YRef
  Bus Element In3 : Inport  Port=2  PortName=Ref  Element=XRef
  Bus Selector1 : BusSelector  OutputSignals=Body.InertFrm.Cg.Ang.phi,Body.InertFrm.Cg.Ang.theta,Body.InertFrm.Cg.Ang.psi  OutputAsBus=on
  Bus Selector10 : BusSelector  OutputSignals=FrntWheels.Wheels.Fx,RearWheels.Wheels.Fx,FrntWheels.Wheels.Fy,RearWheels.Wheels.Fy
  Bus Selector5 : BusSelector  OutputSignals=Steering.Front.WhlAng.FL,Steering.Front.WhlAng.FR,Steering.Rear.WhlAng.RL,Steering.Rear.WhlAng.RR  OutputAsBus=on
  Bus Selector6 : BusSelector  OutputSignals=Body.InertFrm.Geom.Disp.X,Body.InertFrm.Geom.Disp.Y,Body.InertFrm.Geom.Disp.Z  OutputAsBus=on
  Bus Selector7 : BusSelector  OutputSignals=Body.InertFrm.Geom.Vel.Xdot,Body.InertFrm.Geom.Vel.Ydot,Body.InertFrm.Geom.Vel.Zdot  OutputAsBus=on
  Bus Selector9 : BusSelector  OutputSignals=Trans.Info.Eng.EngSpd,EM.EMSpd,Trans.Info.Trans.TransGear
  Bus to Vector{,1..2,4..5} (5 alike) : BusToVector
  Driveline Speed : Subsystem
  Ground1 : Ground
  Mux : Mux  Inputs=3
  Vector Concatenate : Concatenate
  Vector Concatenate1 : Concatenate
  Vector Concatenate2 : Concatenate
  Vehicle XY Plotter : vehdynlibviscommon/Vehicle XY Plot Configuration  extRef=on  extStats=on  extTireF=on  a=PlntVehDstCGFrntAxl  b=PlntVehDstCGRearAxl  w=PlntVehTrckWdth(1)  figBorder=10  bufferSize=1024  velNorm=5  tireFNorm=1000  pltDT=.1
  wires:
  Bus Selector7/1 -> Bus to Vector1/1
  Bus Selector5/1 -> Vehicle XY Plotter/4
  Ground1/1 -> Mux/3
  Bus to Vector1/1 -> Vehicle XY Plotter/3
  Bus Selector1/1 -> Bus to Vector2/1
  Bus Element In1/1 -> Mux/2
  Bus Element In3/1 -> Mux/1
  Mux/1 -> Vehicle XY Plotter/5
  Bus to Vector/1 -> Vehicle XY Plotter/1
  Bus Selector6/1 -> Bus to Vector/1
  Bus to Vector2/1 -> Vehicle XY Plotter/2
  Bus Selector10/1 -> Bus to Vector4/1  "<Fx>"
  Bus Selector10/2 -> Bus to Vector5/1  "<Fx>"
  Bus Selector10/4 -> Vector Concatenate1/2  "<Fy>"
  Vector Concatenate/1 -> Vehicle XY Plotter/7
  Bus Selector10/3 -> Vector Concatenate1/1  "<Fy>"
  Vector Concatenate1/1 -> Vehicle XY Plotter/8
  Bus to Vector4/1 -> Vector Concatenate/1
  Bus to Vector5/1 -> Vector Concatenate/2
  Driveline Speed/1(MaxSpd) -> Vector Concatenate2/1
  Bus Selector9/2 -> Driveline Speed/2(<EMSpd>)  "<EMSpd>"
  Bus Selector9/1 -> Driveline Speed/1(<EngSpd>)  "<EngSpd>"
  Bus Element In2/1 -> Bus Selector5/1, Bus Selector7/1, Bus Selector1/1, Bus Selector6/1, Bus Selector9/1, Bus Selector10/1  "VehFdbk"
  Bus Selector9/3 -> Vector Concatenate2/2  "<TransGear>"
  Vector Concatenate2/1 -> Vehicle XY Plotter/6

== system ConfiguredHevMmVirtualVehicle/Visualization/Vehicle XY Plotter/XY View Ref with One-Axle Trailer ==
  Bus Element In2 : Inport  PortName=VehFdbk
  Bus Element In1 : Inport  Port=2  PortName=Ref  Element=YRef
  Bus Element In3 : Inport  Port=2  PortName=Ref  Element=XRef
  Bus Selector1 : BusSelector  OutputSignals=Body.InertFrm.Cg.Ang.phi,Body.InertFrm.Cg.Ang.theta,Body.InertFrm.Cg.Ang.psi  OutputAsBus=on
  Bus Selector10 : BusSelector  OutputSignals=FrntWheels.Wheels.Fx,RearWheels.Wheels.Fx,FrntWheels.Wheels.Fy,RearWheels.Wheels.Fy,TrlrWheels.Wheels.TireFrame.Fx,TrlrWheels.Wheels.TireFrame.Fy
  Bus Selector16 : BusSelector  OutputSignals=TrlrWheels.Wheels.Steering.WheelAngles  OutputAsBus=on
  Bus Selector2 : BusSelector  OutputSignals=TrlrBody.InertFrm.Geom.Disp.X,TrlrBody.InertFrm.Geom.Disp.Y,TrlrBody.InertFrm.Geom.Disp.Z  OutputAsBus=on
  Bus Selector3 : BusSelector  OutputSignals=TrlrBody.InertFrm.Cg.Ang.phi,TrlrBody.InertFrm.Cg.Ang.theta,TrlrBody.InertFrm.Cg.Ang.psi  OutputAsBus=on
  Bus Selector4 : BusSelector  OutputSignals=TrlrBody.InertFrm.Geom.Vel.Xdot,TrlrBody.InertFrm.Geom.Vel.Ydot,TrlrBody.InertFrm.Geom.Vel.Zdot  OutputAsBus=on
  Bus Selector5 : BusSelector  OutputSignals=Steering.Front.WhlAng.FL,Steering.Front.WhlAng.FR,Steering.Rear.WhlAng.RL,Steering.Rear.WhlAng.RR  OutputAsBus=on
  Bus Selector6 : BusSelector  OutputSignals=Body.InertFrm.Geom.Disp.X,Body.InertFrm.Geom.Disp.Y,Body.InertFrm.Geom.Disp.Z  OutputAsBus=on
  Bus Selector7 : BusSelector  OutputSignals=Body.InertFrm.Geom.Vel.Xdot,Body.InertFrm.Geom.Vel.Ydot,Body.InertFrm.Geom.Vel.Zdot  OutputAsBus=on
  Bus Selector8 : BusSelector  OutputSignals=Trans.Info.Eng.EngSpd,EM.EMSpd,Trans.Info.Trans.TransGear
  Bus to Vector{,1..2,4..9} (9 alike) : BusToVector
  Driveline Speed : Subsystem
  Ground1 : Ground
  Mux : Mux  Inputs=3
  Vector Concatenate : Concatenate
  Vector Concatenate1 : Concatenate
  Vector Concatenate2 : Concatenate
  Vehicle XY Plot Configuration with One-Axle Trailer : vehdynlibviscommon/Vehicle XY Plot Configuration with One-Axle Trailer  extRef=on  extStats=on  extTireF=on  a=PlntVehDstCGFrntAxl  b=PlntVehDstCGRearAxl  w=PlntVehTrckWdth(1)  figBorder=10  bufferSize=1024  velNorm=5  tireFNorm=1000  pltDT=.1
  wires:
  Bus Selector10/4 -> Vector Concatenate1/2  "<Fy>"
  Bus Selector10/1 -> Bus to Vector8/1  "<Fx>"
  Bus Selector10/2 -> Bus to Vector9/1  "<Fx>"
  Bus Selector2/1 -> Bus to Vector4/1
  Vector Concatenate2/1 -> Vehicle XY Plot Configuration with One-Axle Trailer/6
  Bus Selector16/1 -> Bus to Vector7/1
  Bus to Vector/1 -> Vehicle XY Plot Configuration with One-Axle Trailer/1
  Bus to Vector6/1 -> Vehicle XY Plot Configuration with One-Axle Trailer/12
  Ground1/1 -> Mux/3
  Bus Selector7/1 -> Bus to Vector1/1
  Bus Selector4/1 -> Bus to Vector5/1
  Bus to Vector7/1 -> Vehicle XY Plot Configuration with One-Axle Trailer/14
  Bus to Vector4/1 -> Vehicle XY Plot Configuration with One-Axle Trailer/11
  Vector Concatenate1/1 -> Vehicle XY Plot Configuration with One-Axle Trailer/8
  Bus to Vector5/1 -> Vehicle XY Plot Configuration with One-Axle Trailer/13
  Bus Selector10/6 -> Vehicle XY Plot Configuration with One-Axle Trailer/10  "<Fy>"
  Bus Selector3/1 -> Bus to Vector6/1
  Bus Selector6/1 -> Bus to Vector/1
  Mux/1 -> Vehicle XY Plot Configuration with One-Axle Trailer/5
  Bus Selector1/1 -> Bus to Vector2/1
  Bus Element In1/1 -> Mux/2
  Bus Selector10/5 -> Vehicle XY Plot Configuration with One-Axle Trailer/9  "<Fx>"
  Bus Element In3/1 -> Mux/1
  Bus Selector10/3 -> Vector Concatenate1/1  "<Fy>"
  Vector Concatenate/1 -> Vehicle XY Plot Configuration with One-Axle Trailer/7
  Bus Selector5/1 -> Vehicle XY Plot Configuration with One-Axle Trailer/4
  Bus to Vector1/1 -> Vehicle XY Plot Configuration with One-Axle Trailer/3
  Bus to Vector2/1 -> Vehicle XY Plot Configuration with One-Axle Trailer/2
  Bus to Vector8/1 -> Vector Concatenate/1
  Bus to Vector9/1 -> Vector Concatenate/2
  Driveline Speed/1(MaxSpd) -> Vector Concatenate2/1
  Bus Selector8/2 -> Driveline Speed/2(<EMSpd>)  "<EMSpd>"
  Bus Selector8/1 -> Driveline Speed/1(<EngSpd>)  "<EngSpd>"
  Bus Element In2/1 -> Bus Selector10/1, Bus Selector4/1, Bus Selector16/1, Bus Selector3/1, Bus Selector2/1, Bus Selector8/1, Bus Selector5/1, Bus Selector7/1, Bus Selector1/1, Bus Selector6/1  "VehFdbk"
  Bus Selector8/3 -> Vector Concatenate2/2  "<TransGear>"

== system ConfiguredHevMmVirtualVehicle/Driver Commands/Driver Commands/Dashboard Widgets/Widget Sinks ==
  VehFdbk : Inport
  Bus Selector : BusSelector  OutputSignals=Driver.LightsFdbk.HighBeamFdbk,Driver.LightsFdbk.LowBeamFdbk,Driver.LightsFdbk.LeftSignalFdbk,Driver.LightsFdbk.RightSignalFdbk,Driver.LightsFdbk.HazzardFdbk
  Terminator{,1..4} (5 alike) : Terminator
  wires:
  Bus Selector/5 -> Terminator4/1  "<HazzardFdbk>"
  Bus Selector/3 -> Terminator2/1  "<LeftSignalFdbk>"
  Bus Selector/4 -> Terminator3/1  "<RightSignalFdbk>"
  Bus Selector/2 -> Terminator1/1  "<LowBeamFdbk>"
  Bus Selector/1 -> Terminator/1  "<HighBeamFdbk>"
  VehFdbk/1 -> Bus Selector/1

== system ConfiguredHevMmVirtualVehicle/Driver Commands/Driver Commands/Dashboard Widgets/Widget Sources ==
  Accelerator : Constant  Value=0  SampleTime=-1
  Brake : Constant  Value=0  SampleTime=-1
  Bus Assignment : BusAssignment  AssignedSignals=HighBeamCmd,LowBeamCmd,LeftSignalCmd,RightSignalCmd,HazzardCmd
  Bus Creator1 : BusCreator  Inputs=6
  Compare To Constant : simulink/Logic and Bit Operations/Compare To Constant  relop===  const=3  OutDataTypeStr=boolean  ZeroCross=off
  Compare To Constant1 : simulink/Logic and Bit Operations/Compare To Constant  relop===  const=2  OutDataTypeStr=boolean  ZeroCross=off
  Compare To Constant2 : simulink/Logic and Bit Operations/Compare To Constant  relop===  const=-1  OutDataTypeStr=boolean  ZeroCross=off
  Compare To Constant3 : simulink/Logic and Bit Operations/Compare To Constant  relop===  const=1  OutDataTypeStr=boolean  ZeroCross=off
  Data Type Conversion : DataTypeConversion  SaturateOnIntegerOverflow=off  RndMeth=Floor
  Gear : Constant  Value=80  SampleTime=-1
  Hazzard : Constant  Value=0  OutDataTypeStr=boolean
  Headlights : Constant  Value=0
  IgnSwtch : Constant  Value=0
  Scaled Wheel Angle Limit [deg] : Gain  Gain=2*360/90
  Signal Lights : Constant  Value=0
  Signal Specification : SignalSpecification  Unit=1
  Signal Specification1 : SignalSpecification  Unit=1
  Signal Specification2 : SignalSpecification  Unit=1
  Signal Specification3 : SignalSpecification  Unit=deg
  Signal Specification4 : SignalSpecification  OutDataTypeStr=boolean  Unit=1
  Signal Specification5 : SignalSpecification  Unit=rad
  Steer : Constant  Value=0  SampleTime=-1
  To Virtual Bus : SignalConversion  ConversionOutput=Virtual bus  OverrideOpt=off
  Unit Conversion : UnitConversion
  VVCLightsCmd : Constant  Value=0  OutDataTypeStr=Bus: VVCLightsCmdBUS  SampleTime=-1
  Driver : Outport
  wires:
  Scaled Wheel Angle Limit [deg]/1 -> Signal Specification3/1
  Data Type Conversion/1 -> Signal Specification4/1
  Signal Specification4/1 -> Bus Creator1/5  "IgnSwtch"
  Bus Creator1/1 -> Driver/1
  Bus Assignment/1 -> To Virtual Bus/1
  Signal Specification5/1 -> Bus Creator1/1  "SteerCmd"
  Compare To Constant2/1 -> Bus Assignment/4
  Signal Specification3/1 -> Unit Conversion/1
  Gear/1 -> Signal Specification2/1
  To Virtual Bus/1 -> Bus Creator1/6  "LightsCmd"
  Brake/1 -> Signal Specification1/1
  Hazzard/1 -> Bus Assignment/6
  Signal Lights/1 -> Compare To Constant2/1, Compare To Constant3/1
  Signal Specification2/1 -> Bus Creator1/4  "GearCmd"
  Compare To Constant3/1 -> Bus Assignment/5
  VVCLightsCmd/1 -> Bus Assignment/1  "LightsCmd"
  Compare To Constant/1 -> Bus Assignment/2
  Unit Conversion/1 -> Signal Specification5/1
  Accelerator/1 -> Signal Specification/1
  IgnSwtch/1 -> Data Type Conversion/1
  Headlights/1 -> Compare To Constant/1, Compare To Constant1/1
  Steer/1 -> Scaled Wheel Angle Limit [deg]/1
  Signal Specification1/1 -> Bus Creator1/3  "DecelCmd"
  Signal Specification/1 -> Bus Creator1/2  "AccelCmd"
  Compare To Constant1/1 -> Bus Assignment/3

== system ConfiguredHevMmVirtualVehicle/Driver Commands/Driver Commands/Game Wheel Hardware/Paddle Shift ==
  Buttons : Inport
  Add1 : Sum  Inputs=+-+
  Current Gear : UnitDelay  SampleTime=-1  HasFrameUpgradeWarning=on
  Data Type Conversion2 : DataTypeConversion  OutDataTypeStr=double  SaturateOnIntegerOverflow=off  RndMeth=Floor
  Demux2 : Demux  Outputs=2
  Detect Increase2 : simulink/Logic and Bit Operations/Detect Increase  vinit=0.0  OutDataTypeStr=boolean
  Logical Operator1 : Logic  Operator=XOR  Inputs=1  AllPortsSameDT=off  OutDataTypeStr=boolean
  Min/Max Gear : Saturate  UpperLimit=10  LowerLimit=-1
  Selector : Selector  InputPortWidth=32  IndexOptions=Index vector (dialog)  Indices=[5 6]  OutputSizes=1
  Switch2 : Switch  Criteria=u2 > Threshold  SaturateOnIntegerOverflow=off  InputSameDT=off
  Gear : Outport  VectorParamsAs1DForOutWhenUnconnected=off
  wires:
  Selector/1 -> Detect Increase2/1
  Buttons/1 -> Selector/1
  Min/Max Gear/1 -> Switch2/1
  Logical Operator1/1 -> Switch2/2
  Detect Increase2/1 -> Logical Operator1/1, Data Type Conversion2/1
  Data Type Conversion2/1 -> Demux2/1
  Demux2/2 -> Add1/2
  Demux2/1 -> Add1/1
  Switch2/1 -> Current Gear/1, Gear/1  "Gear"
  Current Gear/1 -> Switch2/3, Add1/3
  Add1/1 -> Min/Max Gear/1

== system ConfiguredHevMmVirtualVehicle/Driver Commands/Driver Commands/Game Wheel Hardware/Stick Shift ==
  Buttons : Inport
  Gain : Gain  Gain=[-1 1:6]
  Selector1 : Selector  InputPortWidth=32  IndexOptions=Index vector (dialog)  Indices=[12:18]  OutputSizes=1
  Sum : Sum  Inputs=+
  Gear : Outport  VectorParamsAs1DForOutWhenUnconnected=off
  wires:
  Sum/1 -> Gear/1
  Buttons/1 -> Selector1/1
  Gain/1 -> Sum/1
  Selector1/1 -> Gain/1
